simulink model "hrg_wa_v10_2_modular"  (R2025a)
settings: Solver=FixedStepDiscrete  StartTime=0.0  StopTime=p.duration  FixedStep=p.Ts  RelTol=1e-3
model workspace (MAT data in the model file):
  Ad = [0.987688405123  -5.68131323296e-08  2.48971225508e-05  1.72406495467e-10  2.35500029057e-16  -7.48045553179e-18  2.39085041361e-17  1.59212234261e-22  0  0  0  0; 5.68131323296e-08  0.987688405123  -1.72406495467e-10  2.48971225508e-05  4.70881019476e-18  2.69344781657e-16  -1.59212235008e-22  2.39085041361e-17  0  0  0  0; -982.899001209  -0.00680633562581  0.987672737796  1.37356342331e-05  1.5611837146e-11  -5.09714578103e-13  9.88617178136e-13  1.31942511779e-17  0  0  0  0; 0.00680633562581  -982.899001209  -1.37356342331e-05  0.987672737796  3.12106539235e-13  1.83550880441e-11  -1.31942512097e-17  9.88617178136e-13  0  0  0  0; 0  0  0  0  0.28650479686  0  0  0  0  0  0  0; 0  0  0  0  0  0.352866081459  0  0  0  0  0  0; 943869.866875  6.2854468604  -988.617130951  -0.0131942506432  -1.52887962977e-08  4.97849569843e-10  -9.75634597461e-10  -1.26518662631e-14  0  0  0  0; -6.2854468604  943869.866875  0.0131942506432  -988.617130951  -3.05654153121e-10  -1.79275916498e-08  1.26518662949e-14  -9.75634597462e-10  0  0  0  0; 113668107.931  505.246320907  -239056.237822  -1.59199430864  -2.20191905684e-06  6.98200094534e-08  9.9975990594  -1.46549020767e-12  0.999750031247  0  0  0; -505.246320907  113668107.931  1.59199430864  -239056.237822  -4.4027695682e-08  -2.51395406668e-06  1.46549021355e-12  9.9975990594  0  0.999750031247  0  0; 62170953.3395  1554505.52703  -163920.493963  -4098.88409978  -1.27454644375e-06  4.00156404796e-09  9.50410725413  0.237602681353  0.956612237767  0.0239153059442  0.0432139182638  0; -882829.706009  61193845.2426  2356.91164918  -163353.073245  -7.00440355025e-09  -1.4233603888e-06  -0.139969993764  9.70458623439  -0.0141100303999  0.97829544106  0  0.0591645112941]
  Bd = [1.07541978092e-16  -2.80909408987e-18; 2.15044631223e-18  1.01140599362e-16; 1.17750014529e-11  -3.11685647158e-13; 2.35440509738e-13  1.12226992357e-11; 0.71349520314  0; 0  0.647133918541; -1.10105605369e-08  2.90941885987e-10; -2.20157780066e-10  -1.04757152027e-08; -9.65252715165e-07  2.517993119e-08; -1.93016562843e-08  -9.06591565342e-07; -4.58609339763e-07  1.18833226824e-09; -2.49830556256e-09  -4.18846719335e-07]
  c.detect = [-9972404109.88+545531236.399i  -249309643.885+13636860.8122i; 149494718.172-9008065.32861i  -10364964237.4+624623483.105i]
  c.sample_period_s = 2.5e-05
  c.drive = [1.0677844451e-06-2.20398878536e-07i  -3.17521469995e-08+7.37540079324e-09i; 2.13555769115e-08-4.4075121339e-09i  1.14308554761e-06-2.65485352229e-07i]
  c.nominal_detect = -9999678898.08+46914376.8426i
  p.schema = 'v10.1'
  p.synthetic = 1
  p.f0 = 1000
  p.gamma_intrinsic = 0.314159265359
  p.Cs = 1e-09
  p.G0 = 1e-10
  p.kappa = 1e-06
  p.b = 1.1e-06
  p.Cds = 0
  p.Rs = 1000
  p.B = 0.276990961962
  p.Omega = 0.5
  p.Ts = 2.5e-05
  p.Tc = 0.001
  p.duration = 0.8
  p.charge_target = 1e-11
  p.initial_fraction = 0.3
  p.theta0 = 0.4
  p.Cf = 1e-10
  p.Rf = 1000000000
  p.driver_tau = [2e-05; 2.4e-05]
  p.afe_bw = [20000; 18000]
  p.detect_matrix = [1  0.025; -0.015  1.04]
  p.drive_matrix = [1  -0.03; 0.02  1.08]
  p.split_hz = 0
  p.stiffness_axis = 0.37
  p.damping_half_difference = 0
  p.damping_axis = -0.23
  p.adc_span = 2
  p.adc_bits = 20
  p.dac_span = 2
  p.dac_bits = 18
  p.vmax = 1
  p.agc_bw = 5
  p.quad_bw = 4
  p.pll_gain = 30
  p.max_detune = 30
  p.virtual_rate = 0
  p.virtual_start_min_s = 0.25
  p.virtual_settle_fraction = 0.01
  p.predict_heading = 1
  p.max_heading_rate = 100
  p.virtual_validated_limit = 0.2
  p.min_amplitude_fraction = 0.02
  p.min_linearity = 0.1
  p.max_calibration_condition = 100
  p.max_frame_age = 0.002
  p.calibrate_detection = 1
  p.calibrate_drive = 1
  p.noise_rms_V = 0
  p.noise_seed = 20261030
  x0 = [2.76318298201e-12; 1.16825502693e-12; 0; 0; 0; 0; 0; 0; 0; 0; 0; 0]
libraries: hrg_wa_v10_2_modules x5
Description:
  | V10.2 structural revision inspired by static Gyro.rar module organization. Piezo whole-angle physics and sealed V10.1 controller retained; no SDtoolbox dependency.
settings Model: Creator=11725  LastModifiedBy=11725

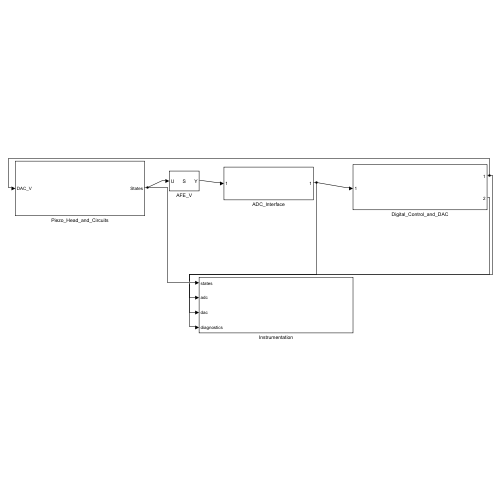
[thumbnail: Simulink's stored preview of the top-level diagram]
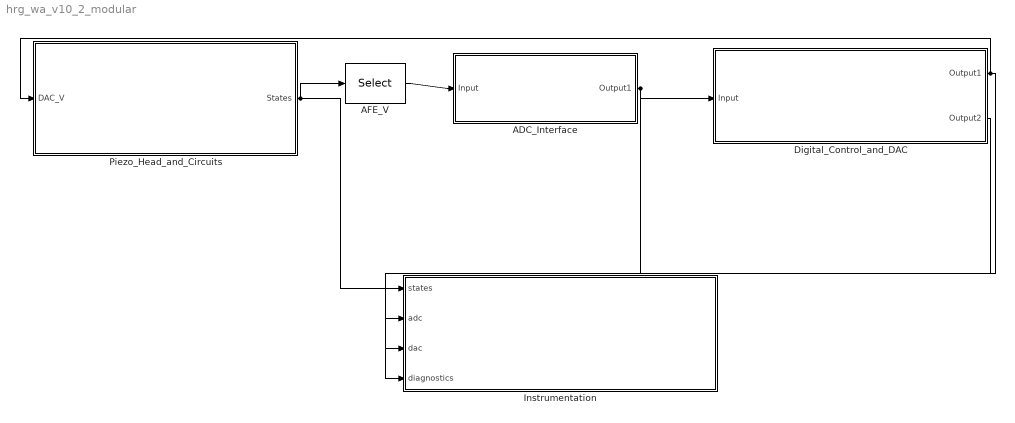
== system hrg_wa_v10_2_modular ==
  ADC_Interface : Subsystem
  AFE_V : Selector  InputPortWidth=12  IndexOptions=Index vector (dialog)  Indices=[11 12]  OutputSizes=1
  Digital_Control_and_DAC : Subsystem  Description=Sealed V10.1 tick: window IQ, validity, calibration, AGC, quadrature, PLL, virtual precession and integer DAC. Algorithm state machine intentionally remains shared for equivalence.
  Instrumentation : Subsystem
  Piezo_Head_and_Circuits : Subsystem  Description=Joint normalized ZOH rows retain reciprocal sensor loading and all within-sample circuit coupling. Every module updates the same sample, no extra delay.
  wires:
  Piezo_Head_and_Circuits/1(States) -> AFE_V/1, Instrumentation/1(states)
  AFE_V/1 -> ADC_Interface/1(Input)
  ADC_Interface/1(Output1) -> Digital_Control_and_DAC/1(Input), Instrumentation/2(adc)
  Digital_Control_and_DAC/1(Output1) -> Piezo_Head_and_Circuits/1(DAC_V), Instrumentation/3(dac)
  Digital_Control_and_DAC/2(Output2) -> Instrumentation/4(diagnostics)

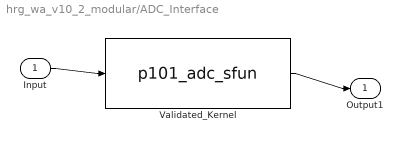
== system hrg_wa_v10_2_modular/ADC_Interface ==
  Input : Inport
  Validated_Kernel : M-S-Function  FunctionName=p101_adc_sfun  Parameters=p
  Output1 : Outport
  wires:
  Input/1 -> Validated_Kernel/1
  Validated_Kernel/1 -> Output1/1

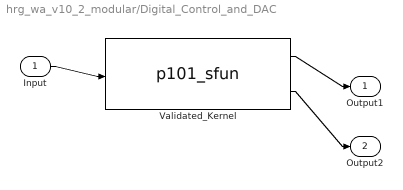
== system hrg_wa_v10_2_modular/Digital_Control_and_DAC ==
  Input : Inport
  Validated_Kernel : M-S-Function  FunctionName=p101_sfun  Parameters=p,c
  Output1 : Outport
  Output2 : Outport  Port=2
  wires:
  Input/1 -> Validated_Kernel/1
  Validated_Kernel/1 -> Output1/1
  Validated_Kernel/2 -> Output2/1

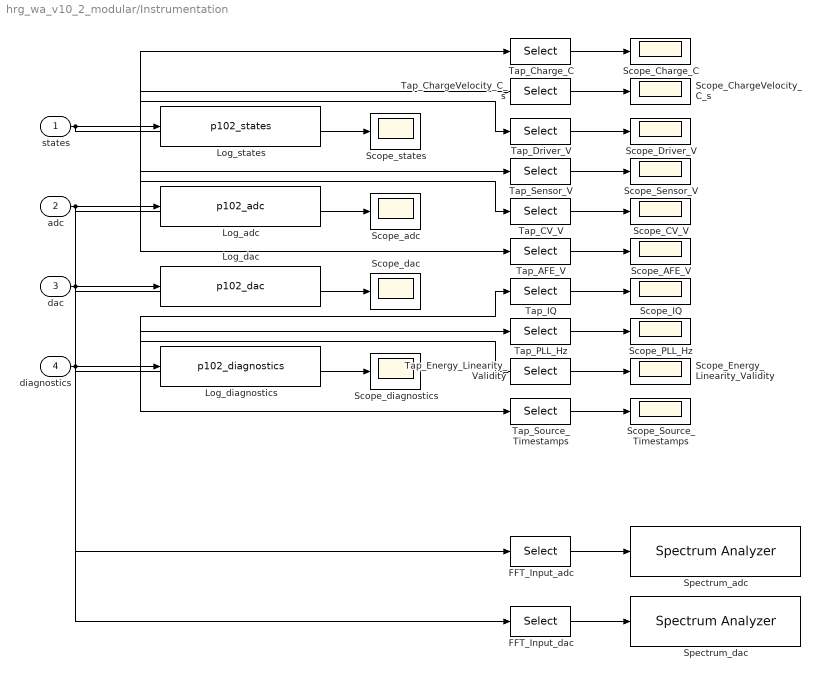
== system hrg_wa_v10_2_modular/Instrumentation ==
  states : Inport
  adc : Inport  Port=2
  dac : Inport  Port=3
  diagnostics : Inport  Port=4
  FFT_Input_adc : Selector  InputPortWidth=4  IndexOptions=Index vector (dialog)  Indices=1  OutputSizes=1
  FFT_Input_dac : Selector  InputPortWidth=2  IndexOptions=Index vector (dialog)  Indices=1  OutputSizes=1
  Log_adc : ToWorkspace  VariableName=p102_adc  SaveFormat=Timeseries  SampleTime=-1
  Log_dac : ToWorkspace  VariableName=p102_dac  SaveFormat=Timeseries  SampleTime=-1
  Log_diagnostics : ToWorkspace  VariableName=p102_diagnostics  SaveFormat=Timeseries  SampleTime=-1
  Log_states : ToWorkspace  VariableName=p102_states  SaveFormat=Timeseries  SampleTime=-1
  Scope_AFE_V : Scope
  Scope_CV_V : Scope
  Scope_ChargeVelocity_C_s : Scope
  Scope_Charge_C : Scope
  Scope_Driver_V : Scope
  Scope_Energy_Linearity_Validity : Scope
  Scope_IQ : Scope
  Scope_PLL_Hz : Scope
  Scope_Sensor_V : Scope
  Scope_Source_Timestamps : Scope
  Scope_adc : Scope
  Scope_dac : Scope
  Scope_diagnostics : Scope
  Scope_states : Scope
  Spectrum_adc : SpectrumAnalyzer  SampleRateSource=Property  SampleRate=1/p.Ts  WindowInvariantSamplesPerUpdate=on  SpectrumUnits=dBV
      settings: OpenAtSimulationStart=off
  Spectrum_dac : SpectrumAnalyzer  SampleRateSource=Property  SampleRate=1/p.Ts  WindowInvariantSamplesPerUpdate=on  SpectrumUnits=dBV
      settings: OpenAtSimulationStart=off
  Tap_AFE_V : Selector  InputPortWidth=12  IndexOptions=Index vector (dialog)  Indices=[11 12]  OutputSizes=1
  Tap_CV_V : Selector  InputPortWidth=12  IndexOptions=Index vector (dialog)  Indices=[9 10]  OutputSizes=1
  Tap_ChargeVelocity_C_s : Selector  InputPortWidth=12  IndexOptions=Index vector (dialog)  Indices=[3 4]  OutputSizes=1
  Tap_Charge_C : Selector  InputPortWidth=12  IndexOptions=Index vector (dialog)  Indices=[1 2]  OutputSizes=1
  Tap_Driver_V : Selector  InputPortWidth=12  IndexOptions=Index vector (dialog)  Indices=[5 6]  OutputSizes=1
  Tap_Energy_Linearity_Validity : Selector  InputPortWidth=18  IndexOptions=Index vector (dialog)  Indices=[6 7 8]  OutputSizes=1
  Tap_IQ : Selector  InputPortWidth=18  IndexOptions=Index vector (dialog)  Indices=[1 2 3 4]  OutputSizes=1
  Tap_PLL_Hz : Selector  InputPortWidth=18  IndexOptions=Index vector (dialog)  Indices=5  OutputSizes=1
  Tap_Sensor_V : Selector  InputPortWidth=12  IndexOptions=Index vector (dialog)  Indices=[7 8]  OutputSizes=1
  Tap_Source_Timestamps : Selector  InputPortWidth=18  IndexOptions=Index vector (dialog)  Indices=[10 11 12 13]  OutputSizes=1
  wires:
  states/1 -> Log_states/1, Scope_states/1, Tap_Charge_C/1, Tap_ChargeVelocity_C_s/1, Tap_Driver_V/1, Tap_Sensor_V/1, Tap_CV_V/1, Tap_AFE_V/1
  adc/1 -> Log_adc/1, Scope_adc/1, FFT_Input_adc/1
  dac/1 -> Log_dac/1, Scope_dac/1, FFT_Input_dac/1
  diagnostics/1 -> Log_diagnostics/1, Scope_diagnostics/1, Tap_IQ/1, Tap_PLL_Hz/1, Tap_Energy_Linearity_Validity/1, Tap_Source_Timestamps/1
  Tap_Charge_C/1 -> Scope_Charge_C/1
  Tap_ChargeVelocity_C_s/1 -> Scope_ChargeVelocity_C_s/1
  Tap_Driver_V/1 -> Scope_Driver_V/1
  Tap_Sensor_V/1 -> Scope_Sensor_V/1
  Tap_CV_V/1 -> Scope_CV_V/1
  Tap_AFE_V/1 -> Scope_AFE_V/1
  Tap_IQ/1 -> Scope_IQ/1
  Tap_PLL_Hz/1 -> Scope_PLL_Hz/1
  Tap_Energy_Linearity_Validity/1 -> Scope_Energy_Linearity_Validity/1
  Tap_Source_Timestamps/1 -> Scope_Source_Timestamps/1
  FFT_Input_adc/1 -> Spectrum_adc/1
  FFT_Input_dac/1 -> Spectrum_dac/1

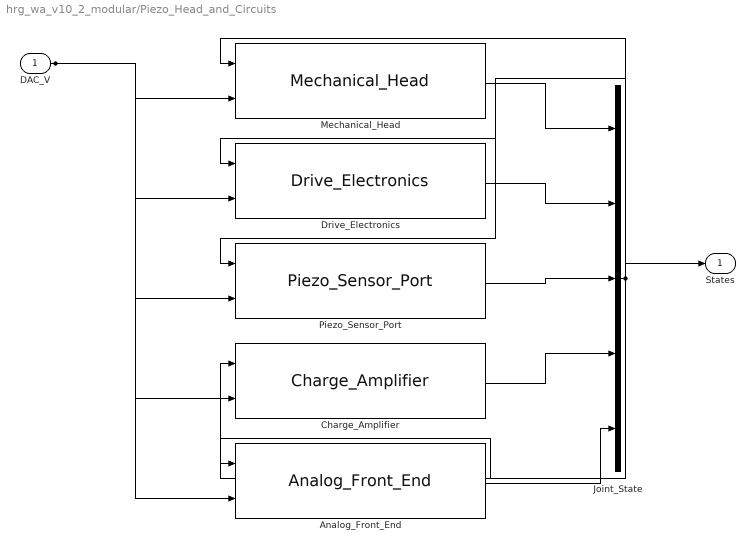
== system hrg_wa_v10_2_modular/Piezo_Head_and_Circuits ==
  DAC_V : Inport
  Analog_Front_End : hrg_wa_v10_2_modules/Analog_Front_End  SystemSampleTime=-1  VariantActivationTime=update diagram  EmptyChoice=off  PassThrough=off  PassThroughVariantControl=(default)  EmptyChoiceVariantControl=(default)  AllowFlexibleInterface=on  Latency=0  AutoFrameSizeCalculation=off
  Charge_Amplifier : hrg_wa_v10_2_modules/Charge_Amplifier  SystemSampleTime=-1  VariantActivationTime=update diagram  EmptyChoice=off  PassThrough=off  PassThroughVariantControl=(default)  EmptyChoiceVariantControl=(default)  AllowFlexibleInterface=on  Latency=0  AutoFrameSizeCalculation=off
  Drive_Electronics : hrg_wa_v10_2_modules/Drive_Electronics  SystemSampleTime=-1  VariantActivationTime=update diagram  EmptyChoice=off  PassThrough=off  PassThroughVariantControl=(default)  EmptyChoiceVariantControl=(default)  AllowFlexibleInterface=on  Latency=0  AutoFrameSizeCalculation=off
  Joint_State : Mux  Inputs=5
  Mechanical_Head : hrg_wa_v10_2_modules/Mechanical_Head  SystemSampleTime=-1  VariantActivationTime=update diagram  EmptyChoice=off  PassThrough=off  PassThroughVariantControl=(default)  EmptyChoiceVariantControl=(default)  AllowFlexibleInterface=on  Latency=0  AutoFrameSizeCalculation=off
  Piezo_Sensor_Port : hrg_wa_v10_2_modules/Piezo_Sensor_Port  SystemSampleTime=-1  VariantActivationTime=update diagram  EmptyChoice=off  PassThrough=off  PassThroughVariantControl=(default)  EmptyChoiceVariantControl=(default)  AllowFlexibleInterface=on  Latency=0  AutoFrameSizeCalculation=off
  States : Outport
  wires:
  Joint_State/1 -> Mechanical_Head/1, Drive_Electronics/1, Piezo_Sensor_Port/1, Charge_Amplifier/1, Analog_Front_End/1, States/1
  DAC_V/1 -> Mechanical_Head/2, Drive_Electronics/2, Piezo_Sensor_Port/2, Charge_Amplifier/2, Analog_Front_End/2
  Mechanical_Head/1 -> Joint_State/1
  Drive_Electronics/1 -> Joint_State/2
  Piezo_Sensor_Port/1 -> Joint_State/3
  Charge_Amplifier/1 -> Joint_State/4
  Analog_Front_End/1 -> Joint_State/5
